simulink model "PV_WIND_BESS_SM_FIXED_R1"  (R2026a)
settings: Solver=ode14x  StopTime=3.2  FixedStep=25e-6  MaxStep=1e-5
InitFcn:
  | setup_v2_paths;init_grid_supported_integration;run(which('init_bess_vsm_r10.m'));
undefined symbols (not defined in the file): Base, Control, Converter, DiscIntNeverNeededParam, Drive, Filter, G, PMSG, V2, Wind
libraries: nesl_utility x50, ee_lib x43, fl_lib x25, simulink x5, sl_discontinuities x1
(part 1 of 4)
Description:
  | Three resources on 10 kV strong synchronous grid. Commissioning candidate only. BESS tie blocked. Wind interface delay 100 us; continuous wind dynamics retained.
settings Model: Creator=fakebob2004  LastModifiedBy=fakebob2004
settings SimscapeCC: SimscapeLogType=none

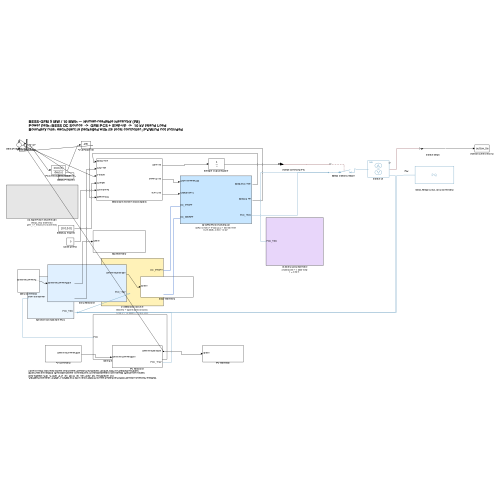
[thumbnail: Simulink's stored preview of the top-level diagram]
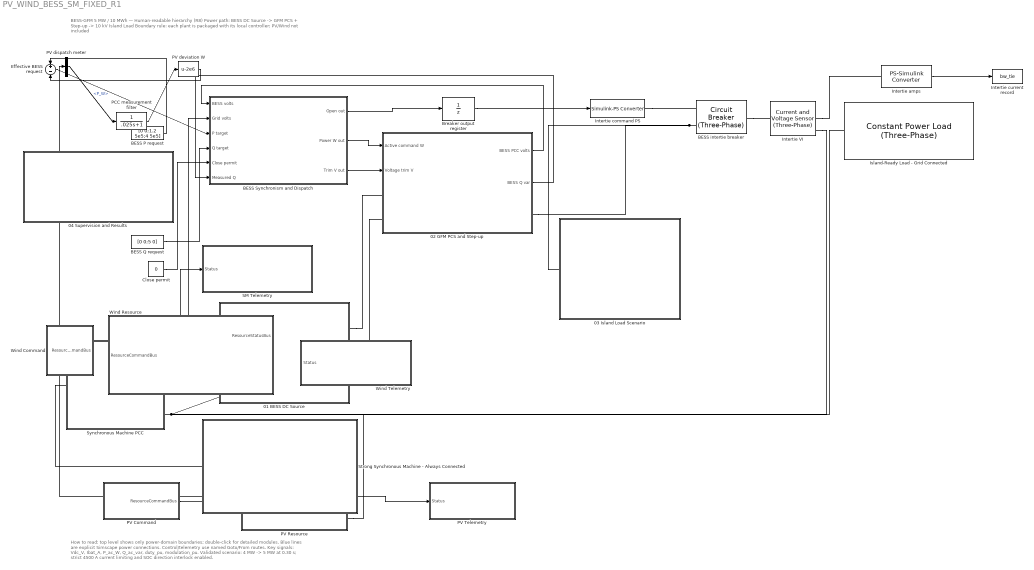
== system PV_WIND_BESS_SM_FIXED_R1 ==
  note: BESS-GFM 5 MW / 10 MWh — Human-readable hierarchy (R8)
      | Power path: BESS DC Source  ->  GFM PCS + Step-up  ->  10 kV Island Load
      | Boundary rule: each plant is packaged with its local controller; PV/Wind not included
  note: How to read: top level shows only power-domain boundaries; double-click for detailed modules.
      | Blue lines are explicit Simscape power connections. Control/telemetry use named Goto/From routes.
      | Key signals: Vdc_V, Ibat_A, P_ac_W, Q_ac_var, duty_pu, modulation_pu.
      | Validated scenario: 4 MW -> 5 MW at 0.30 s; strict 4500 A current limiting and SOC direction interlock enabled.
  01 BESS DC Source : Subsystem
      settings: AttributesFormatString=Battery + bidirectional DC/DC\n1200 V / 10 MWh -> 1500 Vdc
  02 GFM PCS and Step-up : Subsystem
      settings: AttributesFormatString=GFM control + PCS/LCL + transformer\n6.25 MVA, 0.69 / 10 kV
  03 Island Load Scenario : Subsystem
      settings: AttributesFormatString=4 MW base + 1 MW step\nt = 0.30 s
  04 Supervision and Results : Subsystem
      settings: AttributesFormatString=Read-only telemetry\ngfm_r7_result (15 channels)
  BESS P request : FromWorkspace  VariableName=[0 0;1.2 5e5;4 5e5]  Interpolate=off  OutputAfterFinalValue=Holding final value
  BESS Q request : FromWorkspace  VariableName=[0 0;5 0]  Interpolate=off  OutputAfterFinalValue=Holding final value
  BESS Synchronism and Dispatch : Subsystem
  BESS intertie breaker : ee_lib/Switches & Breakers/Circuit Breaker (Three-Phase)  port_option=ee.enum.threePhasePort.composite  control_port_option=ee.enum.controlport.ps  R_closed=0.001 Ohm  G_open=1e-6 1/Ohm  threshold=0.5 V  breaker_behavior=ee.enum.switches.breakerBehavior.zeroCrossingDisable  i_th=1e-8 A
  Breaker output register : UnitDelay  InitialCondition=1  SampleTime=.001
  Close permit : Constant  Value=0
  Effective BESS request : Sum  Inputs=+-
  Intertie VI : ee_lib/Sensors & Transducers/Current and Voltage Sensor (Three-Phase)  port_option=ee.enum.threePhasePort.composite  vMeasurementType=ee.enum.vmeasurement.ll  outputUnit=ee.enum.unit.si  SRated=100e6 A*V  VRated=24e3 V  I_specify=off  I_priority=None  I=[0, 0, 0] A  I_nominal_specify=off  I_nominal_value=1  I_nominal_unit=A  V_specify=off  V_priority=None  V=[0, 0, 0] V  V_nominal_specify=off  V_nominal_value=1  V_nominal_unit=V
  Intertie amps : nesl_utility/PS-Simulink Converter  PhysicalDomain=network_engine_domain  SubClassName=ps_output  LeftPortType=input  RightPortType=output  PseudoPeriodic=off  Frequencies=[]  VectorFormat=inherit  Unit=A  AffineConversion=off
  Intertie command PS : nesl_utility/Simulink-PS Converter  PhysicalDomain=network_engine_domain  SubClassName=ps_input  LeftPortType=input  RightPortType=output  PseudoPeriodic=off  Frequencies=[]  NoiseDistribution=none  NoiseParameters=[]  Unit=V  AffineConversion=off  FilteringAndDerivatives=zero  SimscapeFilterOrder=1  InputFilterTimeConstant=0.001  UdotUserProvided=0
  Intertie current record : ToWorkspace  VariableName=bw_tie  SaveFormat=Timeseries  SampleTime=-1
  Island-Ready Load - Grid Connected : ee_lib/Passive/Constant Power Load (Three-Phase)  port_option=ee.enum.threePhasePort.composite  FRated=50 Hz  active_power=5e6 W  reactive_power=1.5e6 V*A  Vline_rms_min=7000 V  tau=0.01 s  Vline_rms_ini=10000 V  Vang_ini=0 deg  gmin=1e-6 S
  PCC measurement filter : TransferFcn  Numerator=1  Denominator=[.025 1]
  PV Command : Subsystem
  PV Resource : Subsystem
  PV Telemetry : Subsystem
  PV deviation W : Bias  Bias=-2e6  SaturateOnIntegerOverflow=off
  PV dispatch meter : BusSelector  OutputSignals=P_W
  SM Telemetry : Subsystem
  Strong Synchronous Machine - Always Connected : Subsystem
  Synchronous Machine PCC : Subsystem
  Wind Command : Subsystem
  Wind Resource : Subsystem
  Wind Telemetry : Subsystem
  wires:
  02 GFM PCS and Step-up/1(BESS PCC volts) -> BESS Synchronism and Dispatch/1(BESS volts)
  02 GFM PCS and Step-up/2(BESS Q var) -> BESS Synchronism and Dispatch/6(Measured Q)
  BESS Synchronism and Dispatch/2(Power W out) -> 02 GFM PCS and Step-up/1(Active command W)
  Intertie amps/1 -> Intertie current record/1
  BESS Synchronism and Dispatch/1(Open out) -> Breaker output register/1
  Breaker output register/1 -> Intertie command PS/1
  Close permit/1 -> BESS Synchronism and Dispatch/5(Close permit)
  Synchronous Machine PCC/1(PCCMeasurementBus) -> SM Telemetry/1(Status)
  BESS Q request/1 -> BESS Synchronism and Dispatch/4(Q target)
  BESS Synchronism and Dispatch/3(Trim V out) -> 02 GFM PCS and Step-up/2(Voltage trim V)
  Synchronous Machine PCC/2(Phase volts) -> BESS Synchronism and Dispatch/2(Grid volts)
  PV Command/1(ResourceCommandBus) -> PV Resource/1(ResourceCommandBus)
  PV Resource/1(ResourceStatusBus) -> PV Telemetry/1(Status), PV dispatch meter/1
  PV dispatch meter/1 -> PCC measurement filter/1  "<P_W>"
  PCC measurement filter/1 -> PV deviation W/1
  PV deviation W/1 -> Effective BESS request/2
  BESS P request/1 -> Effective BESS request/1
  Effective BESS request/1 -> BESS Synchronism and Dispatch/3(P target)
  Wind Command/1(ResourceCommandBus) -> Wind Resource/1(ResourceCommandBus)
  Wind Resource/1(ResourceStatusBus) -> Wind Telemetry/1(Status)
  connections:
  Intertie VI/RConn2 -- Intertie amps/LConn1
  BESS intertie breaker/RConn1 -- Intertie VI/LConn1
  Intertie command PS/RConn1 -- BESS intertie breaker/LConn1
  01 BESS DC Source/RConn2 -- 02 GFM PCS and Step-up/LConn2
  Strong Synchronous Machine - Always Connected/LConn1 -- Synchronous Machine PCC/LConn1
  01 BESS DC Source/RConn1 -- 02 GFM PCS and Step-up/LConn1
  Intertie VI/RConn3 -- Island-Ready Load - Grid Connected/LConn1 -- PV Resource/RConn1 -- Synchronous Machine PCC/RConn1 -- Wind Resource/RConn1
  02 GFM PCS and Step-up/RConn1 -- 03 Island Load Scenario/LConn1 -- BESS intertie breaker/LConn2

== system PV_WIND_BESS_SM_FIXED_R1/01 BESS DC Source ==
  01 Battery and DC Link : Subsystem
      settings: AttributesFormatString=1200 V / 10 MWh\n1500 V DC link
  02 Bidirectional DC-DC Control : Subsystem
      settings: AttributesFormatString=Vdc PI: 10 Hz\nIbat PI: 300 Hz
  DC_Positive : PMIOPort  Side=Right  ConnectionType=Connection: foundation.electrical.electrical
  DC_Negative : PMIOPort  Port=2  Side=Right  ConnectionType=Connection: foundation.electrical.electrical
  connections:
  02 Bidirectional DC-DC Control/RConn1 -- 01 Battery and DC Link/LConn2
  01 Battery and DC Link/RConn2 -- DC_Negative/RConn1
  DC_Positive/RConn1 -- 01 Battery and DC Link/LConn1

== system PV_WIND_BESS_SM_FIXED_R1/02 GFM PCS and Step-up ==
  Active command W : Inport
  Voltage trim V : Inport  Port=2
  03 GFM Control and Limits : Subsystem
      settings: AttributesFormatString=P-f / Q-V / Virtual Z\nAC limit: 1.20 pu
  04 PCS Filter and Transformer : Subsystem
      settings: AttributesFormatString=6.25 MVA PCS + LCL\n0.69 / 10 kV transformer
  DC_Positive : PMIOPort  Side=Left  ConnectionType=Connection: foundation.electrical.electrical
  DC_Negative : PMIOPort  Port=2  Side=Left  ConnectionType=Connection: foundation.electrical.electrical
  PCC_10kV : PMIOPort  Port=3  Side=Right  ConnectionType=Connection: foundation.electrical.three_phase
  BESS PCC volts : Outport
  BESS Q var : Outport  Port=2
  wires:
  03 GFM Control and Limits/1(GFM modulation reference) -> 04 PCS Filter and Transformer/1(GFM modulation reference)
  04 PCS Filter and Transformer/1(PreSync PCC volts) -> BESS PCC volts/1
  04 PCS Filter and Transformer/2(Measured Q var) -> BESS Q var/1
  Active command W/1 -> 03 GFM Control and Limits/1(Active command W)
  Voltage trim V/1 -> 03 GFM Control and Limits/2(Voltage trim V)
  connections:
  04 PCS Filter and Transformer/RConn3 -- DC_Negative/RConn1
  04 PCS Filter and Transformer/RConn2 -- PCC_10kV/RConn1
  04 PCS Filter and Transformer/RConn1 -- DC_Positive/RConn1
  ?

== system PV_WIND_BESS_SM_FIXED_R1/03 Island Load Scenario ==
  Adjusted_Island_Load : ee_lib/Passive/Constant Power Load (Three-Phase)  port_option=ee.enum.threePhasePort.composite  FRated=G.f0_Hz Hz  active_power=1e4 W  reactive_power=0 V*A  Vline_rms_min=0.70*G.ac.Vll_high_V V  tau=0.01 s  Vline_rms_ini=1e-3 V  Vang_ini=0 deg  gmin=1e-6 S
  Damping neutral : ee_lib/Connectors & References/Grounded Neutral (Three-Phase)  port_option=ee.enum.threePhasePort.composite
  Feeder open request : MinMax  Function=max  Inputs=2
  Load_Step_Command : Step  Time=G.load.step_time_s  InitialValue=1  SampleTime=0
  Load_Step_to_PS : nesl_utility/Simulink-PS Converter  PhysicalDomain=network_engine_domain  SubClassName=ps_input  LeftPortType=input  RightPortType=output  PseudoPeriodic=off  Frequencies=[]  NoiseDistribution=none  NoiseParameters=[]  Unit=V  AffineConversion=off  FilteringAndDerivatives=zero  SimscapeFilterOrder=1  InputFilterTimeConstant=0.001  UdotUserProvided=0
  One_MW_Step_Load : ee_lib/Passive/Constant Power Load (Three-Phase)  port_option=ee.enum.threePhasePort.composite  FRated=G.f0_Hz Hz  active_power=G.load.step_P_W W  reactive_power=G.load.step_Q_var V*A  Vline_rms_min=0.70*G.ac.Vll_high_V V  tau=0.01 s  Vline_rms_ini=1e-3 V  Vang_ini=0 deg  gmin=1e-6 S
  PCC damping RC : ee_lib/Passive/RLC Assemblies/RLC (Three-Phase)  port_option=ee.enum.threePhasePort.composite  component_structure=ee.enum.rlc.structure.SeriesRC  R=10 Ohm  L=1e-3 H  C=1e-6 F  R_parasitic=0 Ohm  G_parasitic=0 1/Ohm  IL_specify=off  IL_priority=High  IL=[0, 0, 0] A  IL_nominal_specify=off  IL_nominal_value=1  IL_nominal_unit=A  VC_specify=off  VC_priority=High  VC=[0, 0, 0] V  VC_nominal_specify=off  VC_nominal_value=1  VC_nominal_unit=V
  Startup feeder hold : Step  Time=.12  InitialValue=1  FinalValue=0  SampleTime=0
  Step_Load_Breaker : ee_lib/Switches & Breakers/Circuit Breaker (Three-Phase)  port_option=ee.enum.threePhasePort.composite  control_port_option=ee.enum.controlport.ps  R_closed=0.001 Ohm  G_open=1e-6 1/Ohm  threshold=0.5 V  breaker_behavior=ee.enum.switches.breakerBehavior.zeroCrossingEnable  i_th=1e-8 A
  PCC_10kV : PMIOPort  Side=Left  ConnectionType=Connection: foundation.electrical.three_phase
  tag scope: R8_05_Island_Load_Scenario_p1_signal=global
  wires:
  Load_Step_Command/1 -> [R8_05_Island_Load_Scenario_p1_signal], Feeder open request/1  "step_breaker_cmd"
  Startup feeder hold/1 -> Feeder open request/2
  Feeder open request/1 -> Load_Step_to_PS/1
  connections:
  Step_Load_Breaker/RConn1 -- One_MW_Step_Load/LConn1
  PCC_10kV/RConn1 -- PCC damping RC/LConn1 -- Adjusted_Island_Load/LConn1 -- Step_Load_Breaker/LConn2
  Load_Step_to_PS/RConn1 -- Step_Load_Breaker/LConn1
  PCC damping RC/RConn1 -- Damping neutral/LConn1

== system PV_WIND_BESS_SM_FIXED_R1/04 Supervision and Results ==
  R7_Result_Mux : Mux  Inputs=15
  R7_Results : ToWorkspace  VariableName=gfm_r7_result  SampleTime=-1
  Time : Clock
  wires:
  [R8_05_Island_Load_Scenario_p1_signal] -> R7_Result_Mux/15
  [R8_03_GFM_Control_and_Limits_p7_signal] -> R7_Result_Mux/14
  R7_Result_Mux/1 -> R7_Results/1
  [R8_03_GFM_Control_and_Limits_p6_signal] -> R7_Result_Mux/13
  [R8_02_Bidirectional_DC_DC_Control_p3_signal] -> R7_Result_Mux/12
  [R8_02_Bidirectional_DC_DC_Control_p2_signal] -> R7_Result_Mux/11
  [R8_01_Battery_and_DC_Link_p3_signal] -> R7_Result_Mux/10
  [R8_03_GFM_Control_and_Limits_p3_signal] -> R7_Result_Mux/9
  [R8_01_Battery_and_DC_Link_p2_signal] -> R7_Result_Mux/8
  [R8_01_Battery_and_DC_Link_p1_signal] -> R7_Result_Mux/7
  [R8_01_Battery_and_DC_Link_p4_signal] -> R7_Result_Mux/6
  [R8_03_GFM_Control_and_Limits_p2_signal] -> R7_Result_Mux/5
  Time/1 -> R7_Result_Mux/1  "time_s"
  [R8_03_GFM_Control_and_Limits_p5_signal] -> R7_Result_Mux/4
  [R8_03_GFM_Control_and_Limits_p1_signal] -> R7_Result_Mux/3
  [R8_03_GFM_Control_and_Limits_p4_signal] -> R7_Result_Mux/2

== system PV_WIND_BESS_SM_FIXED_R1/BESS Synchronism and Dispatch ==
  BESS volts : Inport
  Grid volts : Inport  Port=2
  P target : Inport  Port=3
  Q target : Inport  Port=4
  Close permit : Inport  Port=5
  Measured Q : Inport  Port=6
  Inputs : Mux  Inputs=7
  Open : Fcn  Expr=u(1)
  Power W : Fcn  Expr=u(2)
  Record : ToWorkspace  VariableName=bw_sync  SaveFormat=Timeseries  SampleTime=-1
  Sample : ZeroOrderHold  SampleTime=.001
  State : UnitDelay  InitialCondition=zeros(9,1)  SampleTime=.001
  Synchrocheck and latch : MATLAB Function  TreatAsAtomicUnit=on
  Time : Clock
  Trim V : Fcn  Expr=u(3)
  Open out : Outport
  Power W out : Outport  Port=2
  Trim V out : Outport  Port=3
  wires:
  BESS volts/1 -> Inputs/1
  Grid volts/1 -> Inputs/2
  P target/1 -> Inputs/3
  Q target/1 -> Inputs/4
  Time/1 -> Inputs/5
  Close permit/1 -> Inputs/6
  Measured Q/1 -> Inputs/7
  Inputs/1 -> Sample/1
  Sample/1 -> Synchrocheck and latch/1(u)
  State/1 -> Synchrocheck and latch/2(z)
  Synchrocheck and latch/2(z1) -> State/1
  Synchrocheck and latch/1(y) -> Record/1, Open/1, Power W/1, Trim V/1
  Open/1 -> Open out/1
  Power W/1 -> Power W out/1
  Trim V/1 -> Trim V out/1

== system PV_WIND_BESS_SM_FIXED_R1/PV Command ==
  Command : BusCreator  Inputs=6  OutDataTypeStr=Bus: ResourceCommandBus
  Enable : Constant
  Mode : Constant  Value=0
  P Base : Constant  Value=2000000
  P Increment : Step  Time=2.1  FinalValue=1e6  SampleTime=0
  P Reference : Sum
  Q Reference : Step  Time=10  FinalValue=0  SampleTime=0
  V Reference : Constant  Value=690
  f Reference : Constant  Value=50
  ResourceCommandBus : Outport  OutDataTypeStr=Bus: ResourceCommandBus
  wires:
  Command/1 -> ResourceCommandBus/1
  Mode/1 -> Command/6  "mode"
  Enable/1 -> Command/5  "enable"
  f Reference/1 -> Command/4  "f_ref_Hz"
  V Reference/1 -> Command/3  "V_ref_V"
  Q Reference/1 -> Command/2  "Q_ref_var"
  P Reference/1 -> Command/1  "P_ref_W"
  P Increment/1 -> P Reference/2
  P Base/1 -> P Reference/1

== system PV_WIND_BESS_SM_FIXED_R1/PV Resource ==
  ResourceCommandBus : Inport  OutDataTypeStr=Bus: ResourceCommandBus
  01 PV Array : Subsystem
  02 MPPT Boost and DC Link : Subsystem
  03 Average Grid Converter : Subsystem
  04 Local GFL Control : Subsystem
  05 Filter Transformer and PCC : Subsystem
      settings: AttributesFormatString=independent filter + 0.69/10 kV transformer + PCC sensing
  Command Interface : Subsystem
  Resource Status : Subsystem
  PCC_10kV : PMIOPort  Side=Right  ConnectionType=Connection: foundation.electrical.three_phase
  ResourceStatusBus : Outport  OutDataTypeStr=Bus: ResourceStatusBus
  wires:
  Resource Status/1(Status) -> ResourceStatusBus/1
  Command Interface/3(mode) -> Resource Status/4(mode)
  04 Local GFL Control/2(controlData) -> Resource Status/3(controlData)
  04 Local GFL Control/1(modulationABC) -> 03 Average Grid Converter/1(modulationABC)
  02 MPPT Boost and DC Link/1(sourceData) -> Resource Status/2(sourceData), 04 Local GFL Control/3(sourceData)
  03 Average Grid Converter/1(converterCurrentABC) -> 04 Local GFL Control/2(converterCurrentABC)
  05 Filter Transformer and PCC/1(PCCMeasurementBus) -> Resource Status/1(PCC), 04 Local GFL Control/1(PCCMeasurementBus)
  01 PV Array/1(arrayVI) -> 02 MPPT Boost and DC Link/2(arrayVI)
  Command Interface/2(gridDispatch) -> 04 Local GFL Control/4(dispatch)
  Command Interface/1(sourceDispatch) -> 02 MPPT Boost and DC Link/1(dispatch)
  ResourceCommandBus/1 -> Command Interface/1(Command)
  connections:
  05 Filter Transformer and PCC/RConn1 -- PCC_10kV/RConn1
  03 Average Grid Converter/RConn1 -- 05 Filter Transformer and PCC/LConn1
  02 MPPT Boost and DC Link/RConn2 -- 03 Average Grid Converter/LConn2
  01 PV Array/RConn2 -- 02 MPPT Boost and DC Link/LConn2
  02 MPPT Boost and DC Link/RConn1 -- 03 Average Grid Converter/LConn1
  01 PV Array/RConn1 -- 02 MPPT Boost and DC Link/LConn1

== system PV_WIND_BESS_SM_FIXED_R1/PV Telemetry ==
  Status : Inport
  Fields : BusSelector  OutputSignals=P_W,Q_var,Vpcc_V,frequency_Hz,available_power_W,power_headroom_W,current_limit_factor,energy_state_pu,Vdc_V,control_mode,healthy
  Record : ToWorkspace  VariableName=integration_pv  SaveFormat=Timeseries  SampleTime=-1
  Vector : Mux  Inputs=11
  wires:
  Vector/1 -> Record/1
  Fields/11 -> Vector/11  "<healthy>"
  Fields/10 -> Vector/10  "<control_mode>"
  Fields/9 -> Vector/9  "<Vdc_V>"
  Fields/8 -> Vector/8  "<energy_state_pu>"
  Fields/7 -> Vector/7  "<current_limit_factor>"
  Fields/6 -> Vector/6  "<power_headroom_W>"
  Fields/5 -> Vector/5  "<available_power_W>"
  Fields/4 -> Vector/4  "<frequency_Hz>"
  Fields/3 -> Vector/3  "<Vpcc_V>"
  Fields/2 -> Vector/2  "<Q_var>"
  Fields/1 -> Vector/1  "<P_W>"
  Status/1 -> Fields/1

== system PV_WIND_BESS_SM_FIXED_R1/SM Telemetry ==
  Status : Inport
  Fields : BusSelector  OutputSignals=P_W,Q_var,Vll_rms_V
  Record : ToWorkspace  VariableName=integration_sm  SaveFormat=Timeseries  SampleTime=-1
  Vector : Mux  Inputs=3
  wires:
  Vector/1 -> Record/1
  Fields/3 -> Vector/3  "<Vll_rms_V>"
  Fields/2 -> Vector/2  "<Q_var>"
  Fields/1 -> Vector/1  "<P_W>"
  Status/1 -> Fields/1

== system PV_WIND_BESS_SM_FIXED_R1/Strong Synchronous Machine - Always Connected ==
  Excitation : Constant  Value=1e4*sqrt(2/3)
  Excitation PS : nesl_utility/Simulink-PS Converter  PhysicalDomain=network_engine_domain  SubClassName=ps_input  LeftPortType=input  RightPortType=output  PseudoPeriodic=off  Frequencies=[]  NoiseDistribution=none  NoiseParameters=[]  Unit=V  AffineConversion=off  FilteringAndDerivatives=zero  SimscapeFilterOrder=1  InputFilterTimeConstant=0.001  UdotUserProvided=0
  Governor Speed : Step  Time=10  InitialValue=2*pi*50  FinalValue=2*pi*50  SampleTime=0
  Ideal Governor : fl_lib/Mechanical/Mechanical Sources/Ideal Angular Velocity Source
  Machine Measurements : nesl_utility/PS-Simulink Converter  PhysicalDomain=network_engine_domain  SubClassName=ps_output  LeftPortType=input  RightPortType=output  PseudoPeriodic=off  Frequencies=[]  VectorFormat=inherit  Unit=1  AffineConversion=off
  Machine Record : ToWorkspace  VariableName=integration_machine  SaveFormat=Timeseries  SampleTime=-1
  Mechanical Reference : fl_lib/Mechanical/Rotational Elements/Mechanical Rotational Reference
  Neutral : fl_lib/Electrical/Electrical Elements/Electrical Reference
  Speed PS : nesl_utility/Simulink-PS Converter  PhysicalDomain=network_engine_domain  SubClassName=ps_input  LeftPortType=input  RightPortType=output  PseudoPeriodic=off  Frequencies=[]  NoiseDistribution=none  NoiseParameters=[]  Unit=rad/s  AffineConversion=off  FilteringAndDerivatives=zero  SimscapeFilterOrder=1  InputFilterTimeConstant=0.001  UdotUserProvided=0
  Synchronous Machine : ee_lib/Electromechanical/Synchronous/Simplified Synchronous Machine  port_option=ee.enum.threePhasePort.composite  SRated=100e6 A*V  VRated=10e3 V  FRated=50 Hz  nPolePairs=1  param_unit=ee.enum.unit.si  R_si=0.01 Ohm  L_si=0.001 H  R_pu=0.05  L_pu=0.3  initialization_option=ee.enum.sm.initialization.electrical  source_type=ee.enum.sm.load_flow_source_type.Swing  Vmag0=10e3 V  Vang0=0 deg  Pt0=5e6 A*V  Qt0=1.5e6 A*V  minimum_pu=0.95  phase_search_range=[-inf, inf] deg  gmin=1e-6 S  connection_option=ee.enum.Connection.wye  angular_position_diff_specify=off  angular_position_diff_priority=None  angular_position_diff=0 rad  angular_position_diff_nominal_specify=off  angular_position_diff_nominal_value=1  angular_position_diff_nominal_unit=rad  pu_psid_specify=off  pu_psid_priority=None  pu_psid=0  pu_psid_nominal_specify=off  pu_psid_nominal_value=1  pu_psid_nominal_unit=1  pu_psiq_specify=off  pu_psiq_priority=None  pu_psiq=0  pu_psiq_nominal_specify=off  pu_psiq_nominal_value=1  pu_psiq_nominal_unit=1  pu_psi0_specify=off  pu_psi0_priority=None  pu_psi0=0  pu_psi0_nominal_specify=off  pu_psi0_nominal_value=1  pu_psi0_nominal_unit=1  angular_torque_specify=off  angular_torque_priority=None  angular_torque=0 N*m  angular_torque_nominal_specify=off  angular_torque_nominal_value=1  angular_torque_nominal_unit=N*m  Tmeas=298.15 K  alpha=3.93e-3 1/K  stator_thermal_mass=100 J/K  rotor_thermal_mass=200 J/K  temperatureA_specify=off  temperatureA_priority=High  temperatureA=25 degC  temperatureA_nominal_specify=off  temperatureA_nominal_value=1  temperatureA_nominal_unit=degC  temperatureB_specify=off  temperatureB_priority=High  temperatureB=25 degC  temperatureB_nominal_specify=off  temperatureB_nominal_value=1  temperatureB_nominal_unit=degC  temperatureC_specify=off  temperatureC_priority=High  temperatureC=25 degC  temperatureC_nominal_specify=off  temperatureC_nominal_value=1  temperatureC_nominal_unit=degC  temperatureR_specify=off  temperatureR_priority=High  temperatureR=25 degC  temperatureR_nominal_specify=off  temperatureR_nominal_value=1  temperatureR_nominal_unit=degC
  PCC : PMIOPort  Side=Left  ConnectionType=Connection: foundation.electrical.three_phase
  wires:
  Governor Speed/1 -> Speed PS/1
  Excitation/1 -> Excitation PS/1
  Machine Measurements/1 -> Machine Record/1
  connections:
  PCC/RConn1 -- Synchronous Machine/RConn2
  Synchronous Machine/RConn3 -- Neutral/LConn1
  Excitation PS/RConn1 -- Synchronous Machine/LConn1
  Speed PS/RConn1 -- Ideal Governor/RConn1
  Ideal Governor/LConn1 -- Synchronous Machine/LConn2
  Mechanical Reference/LConn1 -- Ideal Governor/RConn2 -- Synchronous Machine/LConn3
  Synchronous Machine/RConn1 -- Machine Measurements/LConn1

== system PV_WIND_BESS_SM_FIXED_R1/Synchronous Machine PCC ==
  Local PCC Voltage Record : ToWorkspace  VariableName=integration_bus_vabc  SaveFormat=Timeseries  SampleTime=-1
  Nominal Frequency : Constant  Value=V2.PV.rating.f_Hz
  P to Simulink : nesl_utility/PS-Simulink Converter  PhysicalDomain=network_engine_domain  SubClassName=ps_output  LeftPortType=input  RightPortType=output  PseudoPeriodic=off  Frequencies=[]  VectorFormat=inherit  Unit=W  AffineConversion=off
  PCC Measurement : BusCreator  Inputs=6  OutDataTypeStr=Bus: PCCMeasurementBus
  PCC Power Sensor : ee_lib/Sensors & Transducers/Power Sensor (Three-Phase)  port_option=ee.enum.threePhasePort.composite  load_type=ee.enum.passive.type_balanced.balanced  f0=60 Hz
  PCC VI Sensor : ee_lib/Sensors & Transducers/Current and Voltage Sensor (Three-Phase)  port_option=ee.enum.threePhasePort.composite  vMeasurementType=ee.enum.vmeasurement.lg  outputUnit=ee.enum.unit.si  SRated=100e6 A*V  VRated=24e3 V  I_specify=off  I_priority=None  I=[0, 0, 0] A  I_nominal_specify=off  I_nominal_value=1  I_nominal_unit=A  V_specify=off  V_priority=None  V=[0, 0, 0] V  V_nominal_specify=off  V_nominal_value=1  V_nominal_unit=V
  Q to Simulink : nesl_utility/PS-Simulink Converter  PhysicalDomain=network_engine_domain  SubClassName=ps_output  LeftPortType=input  RightPortType=output  PseudoPeriodic=off  Frequencies=[]  VectorFormat=inherit  Unit=W  AffineConversion=off
  Vll RMS : Fcn  Expr=sqrt(u(1)^2+u(2)^2+u(3)^2)
  iabc to Simulink : nesl_utility/PS-Simulink Converter  PhysicalDomain=network_engine_domain  SubClassName=ps_output  LeftPortType=input  RightPortType=output  PseudoPeriodic=off  Frequencies=[]  VectorFormat=inherit  Unit=A  AffineConversion=off
  vabc to Simulink : nesl_utility/PS-Simulink Converter  PhysicalDomain=network_engine_domain  SubClassName=ps_output  LeftPortType=input  RightPortType=output  PseudoPeriodic=off  Frequencies=[]  VectorFormat=inherit  Unit=V  AffineConversion=off
  From Transformer : PMIOPort  Side=Left  ConnectionType=Connection: foundation.electrical.three_phase
  PCC_10kV : PMIOPort  Port=2  Side=Right  ConnectionType=Connection: foundation.electrical.three_phase
  PCCMeasurementBus : Outport  OutDataTypeStr=Bus: PCCMeasurementBus
  Phase volts : Outport  Port=2
  wires:
  PCC Measurement/1 -> PCCMeasurementBus/1
  Nominal Frequency/1 -> PCC Measurement/6  "frequency_Hz"
  Vll RMS/1 -> PCC Measurement/5  "Vll_rms_V"
  Q to Simulink/1 -> PCC Measurement/4  "Q_var"
  P to Simulink/1 -> PCC Measurement/3  "P_W"
  iabc to Simulink/1 -> PCC Measurement/2  "iabc_A"
  vabc to Simulink/1 -> PCC Measurement/1, Local PCC Voltage Record/1, Vll RMS/1, Phase volts/1  "vabc_V"
  connections:
  PCC Power Sensor/LConn3 -- Q to Simulink/LConn1
  PCC Power Sensor/LConn2 -- P to Simulink/LConn1
  PCC VI Sensor/RConn2 -- iabc to Simulink/LConn1
  PCC VI Sensor/RConn1 -- vabc to Simulink/LConn1
  PCC Power Sensor/RConn1 -- PCC_10kV/RConn1
  PCC VI Sensor/RConn3 -- PCC Power Sensor/LConn1
  From Transformer/RConn1 -- PCC VI Sensor/LConn1

== system PV_WIND_BESS_SM_FIXED_R1/Wind Command ==
  Command : BusCreator  Inputs=6  OutDataTypeStr=Bus: ResourceCommandBus
  Enable : Constant
  Mode : Constant  Value=0
  P Base : Constant  Value=2e6
  P Increment : Step  Time=10  FinalValue=0  SampleTime=0
  P Reference : Sum
  Q Reference : Step  Time=10  FinalValue=0  SampleTime=0
  V Reference : Constant  Value=690
  f Reference : Constant  Value=50
  ResourceCommandBus : Outport  OutDataTypeStr=Bus: ResourceCommandBus
  wires:
  Command/1 -> ResourceCommandBus/1
  Mode/1 -> Command/6  "mode"
  Enable/1 -> Command/5  "enable"
  f Reference/1 -> Command/4  "f_ref_Hz"
  V Reference/1 -> Command/3  "V_ref_V"
  Q Reference/1 -> Command/2  "Q_ref_var"
  P Reference/1 -> Command/1  "P_ref_W"
  P Increment/1 -> P Reference/2
  P Base/1 -> P Reference/1

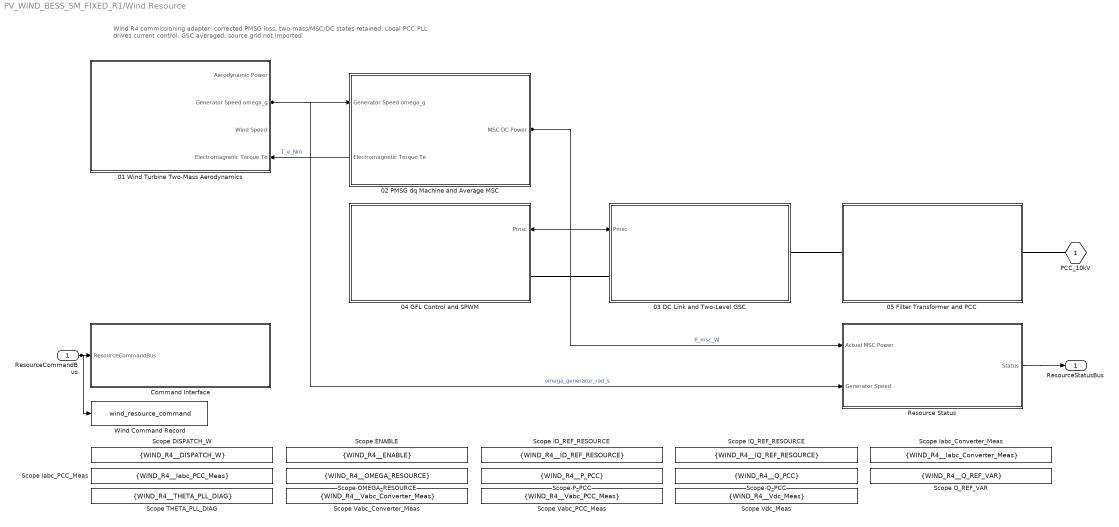
== system PV_WIND_BESS_SM_FIXED_R1/Wind Resource ==
  note: Wind R4 commissioning adapter: corrected PMSG loss, two-mass/MSC/DC states retained. Local PCC PLL drives current control. GSC averaged; source grid not imported.
  ResourceCommandBus : Inport  OutDataTypeStr=Bus: ResourceCommandBus
  01 Wind Turbine Two-Mass Aerodynamics : Subsystem
      settings: PortSchema="{\"entries\":[{\"content\":{\"sides\":[{\"content\":{},\"type\":\"ConnectorPlacement.EquallySpacedRectSide\",\"uuid\":\"d2e99250-fb32-457d-ac2c-6cda9d3cb83e\"},{\"content\":{\"connectorIds\":[\"Out1\",\"Out2\",\"Out3\",\"In1\"],\"side\":\"RIGHT\"},\"type\":\"ConnectorPlacement.EquallySpacedRectSide\",\"uuid\":\"4ed32267-e8b5-4207-a2ca-ef88d31c29b8\"},{\"content\":{\"side\":\"TOP\"},\"type\":\"ConnectorPlacement.EquallySpacedRectSide\",\"uuid\":\"49cb7178-688c-4425-86b9-2e86b87a92d2\"},{\"content\":{\"side\":\"BOTTOM\"},\"type\":\"ConnectorPlacement.EquallySpacedRectSide\",\"uuid\":\"608adf3d-9984-4c8c-8c51-00622b75c623\"}]},\"type\":\"ConnectorPlacement.EquallySpacedConnector\",\"uuid\":\"34aeb2da-84b2-49da-b11b-ab9d51671e98\"}],\"packageUris\":[\"http://schema.mathworks.com/mf0/Connector/R2020b\"],\"version\":\"1.0\"}"
  02 PMSG dq Machine and Average MSC : Subsystem
      settings: PortSchema="{\"entries\":[{\"content\":{\"sides\":[{\"content\":{\"connectorIds\":[\"In1\",\"Out1\"]},\"type\":\"ConnectorPlacement.EquallySpacedRectSide\",\"uuid\":\"48609cb7-5ec2-40c8-9ad6-e417a7f110fc\"},{\"content\":{\"connectorIds\":[\"Out2\"],\"side\":\"RIGHT\"},\"type\":\"ConnectorPlacement.EquallySpacedRectSide\",\"uuid\":\"fe5978ba-7578-46e7-b8bd-8d766a317898\"},{\"content\":{\"side\":\"TOP\"},\"type\":\"ConnectorPlacement.EquallySpacedRectSide\",\"uuid\":\"e50b8460-8f11-49ca-af82-a50e0a9897ac\"},{\"content\":{\"side\":\"BOTTOM\"},\"type\":\"ConnectorPlacement.EquallySpacedRectSide\",\"uuid\":\"e858deaf-0aa3-40bd-b11b-e0cbf70df614\"}]},\"type\":\"ConnectorPlacement.EquallySpacedConnector\",\"uuid\":\"52c7dc97-51f1-4b4e-ac97-f0f7de231d0c\"}],\"packageUris\":[\"http://schema.mathworks.com/mf0/Connector/R2020b\"],\"version\":\"1.0\"}"
  03 DC Link and Two-Level GSC : Subsystem
  04 GFL Control and SPWM : Subsystem
      settings: PortSchema="{\"entries\":[{\"content\":{\"sides\":[{\"content\":{},\"type\":\"ConnectorPlacement.EquallySpacedRectSide\",\"uuid\":\"789c4a44-46fc-465a-8542-50ccb2941023\"},{\"content\":{\"connectorIds\":[\"In1\",\"RConn1\"],\"side\":\"RIGHT\"},\"type\":\"ConnectorPlacement.EquallySpacedRectSide\",\"uuid\":\"a82b7ba7-9d1b-4671-ba15-c7f8930ba494\"},{\"content\":{\"side\":\"TOP\"},\"type\":\"ConnectorPlacement.EquallySpacedRectSide\",\"uuid\":\"e4af03d8-b6a4-4af9-a989-7508e05466ea\"},{\"content\":{\"side\":\"BOTTOM\"},\"type\":\"ConnectorPlacement.EquallySpacedRectSide\",\"uuid\":\"c53f6650-4639-4f00-bd86-9fb4ea7f36eb\"}]},\"type\":\"ConnectorPlacement.EquallySpacedConnector\",\"uuid\":\"b3a75c1a-8bf0-4d48-a914-c2377b7f5048\"}],\"packageUris\":[\"http://schema.mathworks.com/mf0/Connector/R2020b\"],\"version\":\"1.0\"}"
  05 Filter Transformer and PCC : Subsystem
  Command Interface : Subsystem
  Resource Status : Subsystem
  Scope DISPATCH_W : GotoTagVisibility  GotoTag=WIND_R4__DISPATCH_W
  Scope ENABLE : GotoTagVisibility  GotoTag=WIND_R4__ENABLE
  Scope ID_REF_RESOURCE : GotoTagVisibility  GotoTag=WIND_R4__ID_REF_RESOURCE
  Scope IQ_REF_RESOURCE : GotoTagVisibility  GotoTag=WIND_R4__IQ_REF_RESOURCE
  Scope Iabc_Converter_Meas : GotoTagVisibility  GotoTag=WIND_R4__Iabc_Converter_Meas
  Scope Iabc_PCC_Meas : GotoTagVisibility  GotoTag=WIND_R4__Iabc_PCC_Meas
  Scope OMEGA_RESOURCE : GotoTagVisibility  GotoTag=WIND_R4__OMEGA_RESOURCE
  Scope P_PCC : GotoTagVisibility  GotoTag=WIND_R4__P_PCC
  Scope Q_PCC : GotoTagVisibility  GotoTag=WIND_R4__Q_PCC
  Scope Q_REF_VAR : GotoTagVisibility  GotoTag=WIND_R4__Q_REF_VAR
  Scope THETA_PLL_DIAG : GotoTagVisibility  GotoTag=WIND_R4__THETA_PLL_DIAG
  Scope Vabc_Converter_Meas : GotoTagVisibility  GotoTag=WIND_R4__Vabc_Converter_Meas
  Scope Vabc_PCC_Meas : GotoTagVisibility  GotoTag=WIND_R4__Vabc_PCC_Meas
  Scope Vdc_Meas : GotoTagVisibility  GotoTag=WIND_R4__Vdc_Meas
  Wind Command Record : ToWorkspace  VariableName=wind_resource_command  SaveFormat=Timeseries  SampleTime=-1
  PCC_10kV : PMIOPort  Side=Right  ConnectionType=Connection: foundation.electrical.three_phase
  ResourceStatusBus : Outport  OutDataTypeStr=Bus: ResourceStatusBus
  wires:
  Resource Status/1(Status) -> ResourceStatusBus/1
  ResourceCommandBus/1 -> Wind Command Record/1, Command Interface/1(ResourceCommandBus)
  02 PMSG dq Machine and Average MSC/2(MSC DC Power) -> Resource Status/1(Actual MSC Power), 04 GFL Control and SPWM/1(Pmsc), 03 DC Link and Two-Level GSC/1(Pmsc)  "P_msc_W"
  02 PMSG dq Machine and Average MSC/1(Electromagnetic Torque Te) -> 01 Wind Turbine Two-Mass Aerodynamics/1(Electromagnetic Torque Te)  "T_e_Nm"
  01 Wind Turbine Two-Mass Aerodynamics/2(Generator Speed omega_g) -> Resource Status/2(Generator Speed), 02 PMSG dq Machine and Average MSC/1(Generator Speed omega_g)  "omega_generator_rad_s"
  connections:
  05 Filter Transformer and PCC/RConn1 -- PCC_10kV/RConn1
  03 DC Link and Two-Level GSC/RConn1 -- 05 Filter Transformer and PCC/LConn1
  04 GFL Control and SPWM/RConn1 -- 03 DC Link and Two-Level GSC/LConn1

== system PV_WIND_BESS_SM_FIXED_R1/Wind Telemetry ==
  Status : Inport
  Fields : BusSelector  OutputSignals=P_W,Q_var,Vpcc_V,frequency_Hz,available_power_W,power_headroom_W,current_limit_factor,energy_state_pu,Vdc_V,control_mode,healthy
  Record : ToWorkspace  VariableName=integration_wind  SaveFormat=Timeseries  SampleTime=-1
  Vector : Mux  Inputs=11
  wires:
  Vector/1 -> Record/1
  Fields/11 -> Vector/11  "<healthy>"
  Fields/10 -> Vector/10  "<control_mode>"
  Fields/9 -> Vector/9  "<Vdc_V>"
  Fields/8 -> Vector/8  "<energy_state_pu>"
  Fields/7 -> Vector/7  "<current_limit_factor>"
  Fields/6 -> Vector/6  "<power_headroom_W>"
  Fields/5 -> Vector/5  "<available_power_W>"
  Fields/4 -> Vector/4  "<frequency_Hz>"
  Fields/3 -> Vector/3  "<Vpcc_V>"
  Fields/2 -> Vector/2  "<Q_var>"
  Fields/1 -> Vector/1  "<P_W>"
  Status/1 -> Fields/1

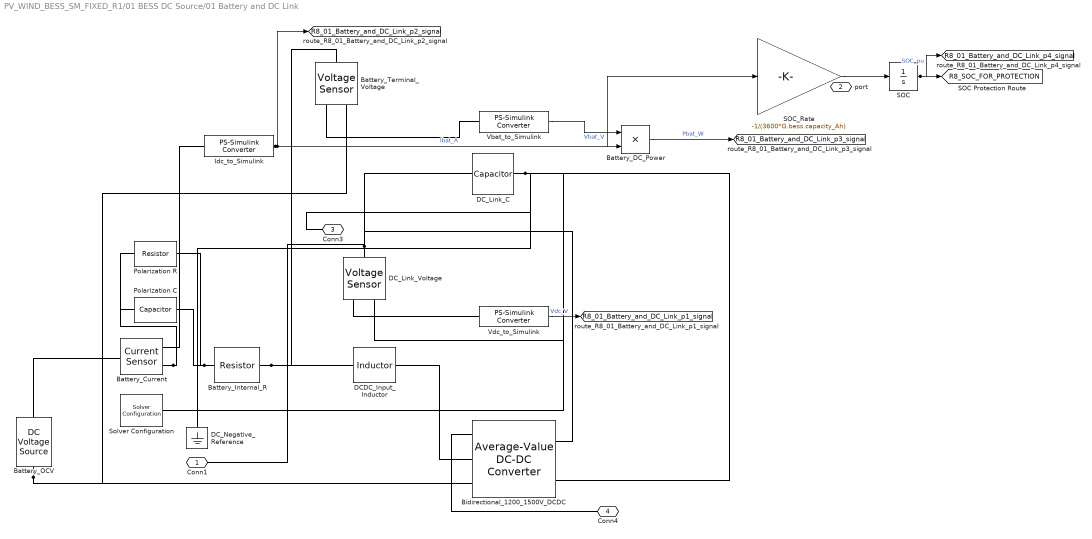
== system PV_WIND_BESS_SM_FIXED_R1/01 BESS DC Source/01 Battery and DC Link ==
  Battery_Current : fl_lib/Electrical/Electrical Sensors/Current Sensor
  Battery_DC_Power : Product
  Battery_Internal_R : fl_lib/Electrical/Electrical Elements/Resistor  R=G.r9.R0 Ohm  i_specify=off  i_priority=None  i=0 A  i_nominal_specify=off  i_nominal_value=1  i_nominal_unit=A  v_specify=off  v_priority=None  v=0 V  v_nominal_specify=off  v_nominal_value=1  v_nominal_unit=V
  Battery_OCV : fl_lib/Electrical/Electrical Sources/DC Voltage Source  v0=G.dc.Vbattery_V V
  Battery_Terminal_Voltage : fl_lib/Electrical/Electrical Sensors/Voltage Sensor
  Bidirectional_1200_1500V_DCDC : ee_lib/Semiconductors & Converters/Converters/Average-Value DC-DC Converter  implementation_option=ee.enum.converters.implementation.behavioral  converter_type=ee.enum.converters.dcdctype.buckboost  control_option=ee.enum.converters.controlinput.dutycycle  efficiency_option=ee.enum.converters.efficiency.constant  efficiency_fixed=G.dc.dcdc_efficiency_pct  i_vec=[0, 2, 5] A  efficiency_vec=[90, 95, 98]  Lf=1e-6 H  Rl=0 Ohm  Cf=1e-7 F  Rc=1e-6 Ohm  iL_specify=off  iL_priority=High  iL=0 A  iL_nominal_specify=off  iL_nominal_value=1  iL_nominal_unit=A  vc_specify=off  vc_priority=High  vc=0 V  vc_nominal_specify=off  vc_nominal_value=1  vc_nominal_unit=V
  DCDC_Input_Inductor : fl_lib/Electrical/Electrical Elements/Inductor  l=G.dcdc.L_H H  r=0 Ohm  g=1e-9 1/Ohm  i_specify=on  i_priority=None  i=G.dcdc.Iref_initial_A A  i_nominal_specify=off  i_nominal_value=1  i_nominal_unit=A  v_specify=off  v_priority=None  v=0 V  v_nominal_specify=off  v_nominal_value=1  v_nominal_unit=V  i_L_specify=off  i_L_priority=High  i_L=0 A  i_L_nominal_specify=off  i_L_nominal_value=1  i_L_nominal_unit=A
  DC_Link_C : fl_lib/Electrical/Electrical Elements/Capacitor  c=G.dc.Cdc_F F  r=1e-6 Ohm  g=0 1/Ohm  i_specify=off  i_priority=None  i=0 A  i_nominal_specify=off  i_nominal_value=1  i_nominal_unit=A  v_specify=off  v_priority=None  v=0 V  v_nominal_specify=off  v_nominal_value=1  v_nominal_unit=V  vc_specify=on  vc_priority=High  vc=G.dc.Vdc_ref_V V  vc_nominal_specify=off  vc_nominal_value=1  vc_nominal_unit=V
  DC_Link_Voltage : fl_lib/Electrical/Electrical Sensors/Voltage Sensor
  DC_Negative_Reference : fl_lib/Electrical/Electrical Elements/Electrical Reference
  Idc_to_Simulink : nesl_utility/PS-Simulink Converter  PhysicalDomain=network_engine_domain  SubClassName=ps_output  LeftPortType=input  RightPortType=output  PseudoPeriodic=off  Frequencies=[]  VectorFormat=inherit  Unit=A  AffineConversion=off
  Polarization C : fl_lib/Electrical/Electrical Elements/Capacitor  c=G.r9.tau/G.r9.Rp F  r=1e-6 Ohm  g=0 1/Ohm  i_specify=off  i_priority=None  i=0 A  i_nominal_specify=off  i_nominal_value=1  i_nominal_unit=A  v_specify=off  v_priority=None  v=0 V  v_nominal_specify=off  v_nominal_value=1  v_nominal_unit=V  vc_specify=on  vc_priority=High  vc=0 V  vc_nominal_specify=off  vc_nominal_value=1  vc_nominal_unit=V
  Polarization R : fl_lib/Electrical/Electrical Elements/Resistor  R=G.r9.Rp Ohm  i_specify=off  i_priority=None  i=0 A  i_nominal_specify=off  i_nominal_value=1  i_nominal_unit=A  v_specify=off  v_priority=None  v=0 V  v_nominal_specify=off  v_nominal_value=1  v_nominal_unit=V
  SOC : Integrator  InitialCondition=G.bess.SOC0  LimitOutput=on  UpperSaturationLimit=G.bess.SOC_max  LowerSaturationLimit=G.bess.SOC_min
  SOC_Rate : Gain  Gain=-1/(3600*G.bess.capacity_Ah)
  Solver Configuration : nesl_utility/Solver Configuration  PhysicalDomain=network_engine_domain  SubClassName=solver  LeftPortType=input  RightPortType=generic  Tones=[]  Harmonics=[]  SimulateNoise=off  Profile=off  UseLocalSampling=off  EnableSwitchedLinearOptims=on  FrequencyDomain=off  UseCCode=off  RelTol=0.001  AbsTol=0.001  MinStep=1e-09  ToWorkspace=off  RevertToSquareIcSolve=off  NumHomotopyIterations=100  PhasorMode=off  PhasorModeNumHarmonics=1  ConsistencySolver=NEWTON_XTOL_AFTER_FTOL  CanonicalOrdering=CANONICAL  OptimizeIntermediates=OPTIMIZED  IndexReductionMethod=DerivativeReplacement  DoDC=off  ResidualTolerance=1e-09  ConsistencyTolSource=GLOBAL  ConsistencyAbsTol=0.001  ConsistencyRelTol=0.001  ConsistencyTolFactor=0.001  UseLocalSolver=on  LocalSolverChoice=NE_BACKWARD_EULER_ADVANCER  ResolveIndetEquations=on  FunctionEvalNumThread=1  LocalSolverSampleTime=25e-6  DoFixedCost=off  MaxNonlinIter=3  MaxModeIter=2  ComputeImpulses=off  ImpulseIterations=2  LinearAlgebra=auto  LinearAlgebraNumThread=0  EquationFormulation=NE_TIME_EF  DelaysMemoryBudget=1024  AutomaticFiltering=on  FilteringTimeConstant=0.001  PartitionStorageMethod=AS_NEEDED  PartitionMemoryBudget=1024  PartitionMethod=ROBUST  MultibodyUseLocalSolver=off  MultibodyLocalSolverChoice=ODE1  MultibodyLocalSolverSampleTime=0.001
  Vbat_to_Simulink : nesl_utility/PS-Simulink Converter  PhysicalDomain=network_engine_domain  SubClassName=ps_output  LeftPortType=input  RightPortType=output  PseudoPeriodic=off  Frequencies=[]  VectorFormat=inherit  Unit=V  AffineConversion=off
  Vdc_to_Simulink : nesl_utility/PS-Simulink Converter  PhysicalDomain=network_engine_domain  SubClassName=ps_output  LeftPortType=input  RightPortType=output  PseudoPeriodic=off  Frequencies=[]  VectorFormat=inherit  Unit=V  AffineConversion=off
  Conn1 : PMIOPort  Side=Left
  port : PMIOPort  Port=2  Side=Right
  Conn3 : PMIOPort  Port=3  Side=Right
  Conn4 : PMIOPort  Port=4  Side=Left
  tag scope: R8_01_Battery_and_DC_Link_p1_signal=global, R8_01_Battery_and_DC_Link_p2_signal=global, R8_01_Battery_and_DC_Link_p3_signal=global, R8_01_Battery_and_DC_Link_p4_signal=global, R8_SOC_FOR_PROTECTION=global
  wires:
  SOC/1 -> [R8_01_Battery_and_DC_Link_p4_signal], [R8_SOC_FOR_PROTECTION]  "SOC_pu"
  Battery_DC_Power/1 -> [R8_01_Battery_and_DC_Link_p3_signal]  "Pbat_W"
  Vbat_to_Simulink/1 -> Battery_DC_Power/1  "Vbat_V"
  Vdc_to_Simulink/1 -> [R8_01_Battery_and_DC_Link_p1_signal]  "Vdc_V"
  SOC_Rate/1 -> SOC/1
  Idc_to_Simulink/1 -> [R8_01_Battery_and_DC_Link_p2_signal], Battery_DC_Power/2, SOC_Rate/1  "Ibat_A"
  connections:
  Conn4/RConn1 -- Bidirectional_1200_1500V_DCDC/LConn1
  DC_Link_Voltage/LConn1 -- Bidirectional_1200_1500V_DCDC/RConn1 -- DC_Link_C/LConn1 -- Conn1/RConn1
  Battery_Terminal_Voltage/RConn1 -- Vbat_to_Simulink/LConn1
  DC_Link_Voltage/RConn1 -- Vdc_to_Simulink/LConn1
  Battery_Internal_R/RConn1 -- DCDC_Input_Inductor/LConn1 -- Battery_Terminal_Voltage/LConn1
  DCDC_Input_Inductor/RConn1 -- Bidirectional_1200_1500V_DCDC/LConn2
  Battery_Current/RConn1 -- Idc_to_Simulink/LConn1
  Battery_OCV/LConn1 -- Battery_Current/LConn1
  DC_Negative_Reference/LConn1 -- DC_Link_C/RConn1 -- Bidirectional_1200_1500V_DCDC/RConn2 -- DC_Link_Voltage/RConn2 -- Conn3/RConn1 -- Solver Configuration/RConn1
  Battery_OCV/RConn1 -- Battery_Terminal_Voltage/RConn2 -- Bidirectional_1200_1500V_DCDC/LConn3
  Polarization R/LConn1 -- Battery_Current/RConn2 -- Polarization C/LConn1
  Battery_Internal_R/LConn1 -- Polarization R/RConn1 -- Polarization C/RConn1

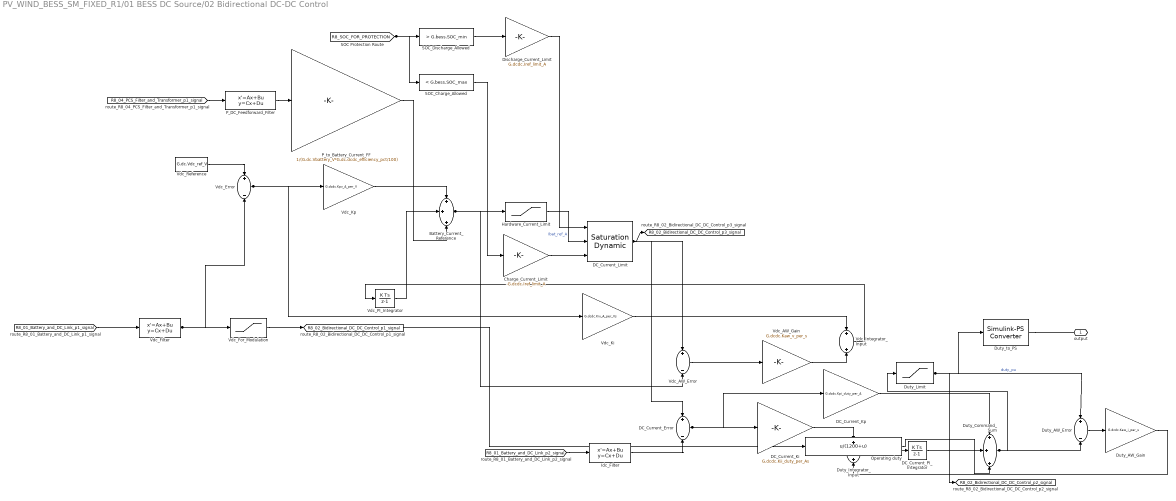
== system PV_WIND_BESS_SM_FIXED_R1/01 BESS DC Source/02 Bidirectional DC-DC Control ==
  Battery_Current_Reference : Sum  Inputs=+++
  Charge_Current_Limit : Gain  Gain=-G.dcdc.Iref_limit_A
  DC_Current_Error : Sum  Inputs=+-
  DC_Current_Ki : Gain  Gain=G.dcdc.Kii_duty_per_As
  DC_Current_Kp : Gain  Gain=G.dcdc.Kpi_duty_per_A
  DC_Current_Limit : sl_discontinuities/Saturation Dynamic  OutMin=[]  OutMax=[]  OutDataTypeStr=Inherit: Same as second input  OutDataType=fixdt(1, 16)  OutScaling=2^-10  DoSatur=off
      settings: LibrarySourceBlock=|
      | simulink/Discontinuities/Saturation
      | Dynamic
  DC_Current_PI_Integrator : DiscreteIntegrator  SampleTime=100e-6  ICPrevOutput=DiscIntNeverNeededParam  ICPrevScaledInput=DiscIntNeverNeededParam
  Discharge_Current_Limit : Gain  Gain=G.dcdc.Iref_limit_A
  Duty_AW_Error : Sum  Inputs=+-
  Duty_AW_Gain : Gain  Gain=G.dcdc.Kaw_i_per_s
  Duty_Command_Sum : Sum  Inputs=+++
  Duty_Integrator_Input : Sum
  Duty_Limit : Saturate  UpperLimit=G.dcdc.duty_max  LowerLimit=G.dcdc.duty_min
  Duty_to_PS : nesl_utility/Simulink-PS Converter  PhysicalDomain=network_engine_domain  SubClassName=ps_input  LeftPortType=input  RightPortType=output  PseudoPeriodic=off  Frequencies=[]  NoiseDistribution=none  NoiseParameters=[]  Unit=1  AffineConversion=off  FilteringAndDerivatives=zero  SimscapeFilterOrder=1  InputFilterTimeConstant=0.001  UdotUserProvided=0
  Hardware_Current_Limit : Saturate  UpperLimit=G.dcdc.Iref_limit_A  LowerLimit=-G.dcdc.Iref_limit_A
  Idc_Filter : StateSpace  A=-1/G.dcdc.current_sensor_s  B=1/G.dcdc.current_sensor_s  D=0  InitialCondition=G.dcdc.Iref_initial_A
  Operating duty : Fcn  Expr=u/(1200+u)
  P_DC_Feedforward_Filter : StateSpace  A=-1/G.dcdc.power_ff_filter_s  B=1/G.dcdc.power_ff_filter_s  D=0  InitialCondition=0
  P_to_Battery_Current_FF : Gain  Gain=1/(G.dc.Vbattery_V*G.dc.dcdc_efficiency_pct/100)
  SOC_Charge_Allowed : simulink/Logic and Bit Operations/Compare To Constant  relop=<  const=G.bess.SOC_max  OutDataTypeStr=boolean
  SOC_Discharge_Allowed : simulink/Logic and Bit Operations/Compare To Constant  relop=>  const=G.bess.SOC_min  OutDataTypeStr=boolean
  Vdc_AW_Error : Sum  Inputs=+-
  Vdc_AW_Gain : Gain  Gain=G.dcdc.Kaw_v_per_s
  Vdc_Error : Sum  Inputs=+-
  Vdc_Filter : StateSpace  A=-1/G.control.Vdc_filter_s  B=1/G.control.Vdc_filter_s  D=0  InitialCondition=G.dc.Vdc_ref_V
  Vdc_For_Modulation : Saturate  UpperLimit=2000  LowerLimit=500
  Vdc_Integrator_Input : Sum
  Vdc_Ki : Gain  Gain=G.dcdc.Kiv_A_per_Vs
  Vdc_Kp : Gain  Gain=G.dcdc.Kpv_A_per_V
  Vdc_PI_Integrator : DiscreteIntegrator  SampleTime=100e-6  ICPrevOutput=DiscIntNeverNeededParam  ICPrevScaledInput=DiscIntNeverNeededParam
  Vdc_Reference : Constant  Value=G.dc.Vdc_ref_V
  output : PMIOPort  Side=Right
  tag scope: R8_02_Bidirectional_DC_DC_Control_p1_signal=global, R8_02_Bidirectional_DC_DC_Control_p2_signal=global, R8_02_Bidirectional_DC_DC_Control_p3_signal=global
  wires:
  Duty_AW_Gain/1 -> Duty_Integrator_Input/2
  Duty_Limit/1 -> [R8_02_Bidirectional_DC_DC_Control_p2_signal], Duty_AW_Error/1, Duty_to_PS/1  "duty_pu"
  Duty_Integrator_Input/1 -> DC_Current_PI_Integrator/1
  DC_Current_Error/1 -> DC_Current_Ki/1, DC_Current_Kp/1
  Idc_Filter/1 -> DC_Current_Error/2
  Discharge_Current_Limit/1 -> DC_Current_Limit/1
  Vdc_Ki/1 -> Vdc_Integrator_Input/1
  SOC_Charge_Allowed/1 -> Charge_Current_Limit/1
  DC_Current_Limit/1 -> [R8_02_Bidirectional_DC_DC_Control_p3_signal], DC_Current_Error/1, Vdc_AW_Error/1
  [R8_01_Battery_and_DC_Link_p2_signal] -> Idc_Filter/1
  Vdc_AW_Error/1 -> Vdc_AW_Gain/1
  Charge_Current_Limit/1 -> DC_Current_Limit/3
  Hardware_Current_Limit/1 -> DC_Current_Limit/2  "Ibat_ref_A"
  Vdc_Integrator_Input/1 -> Vdc_PI_Integrator/1
  Battery_Current_Reference/1 -> Hardware_Current_Limit/1, Vdc_AW_Error/2
  DC_Current_PI_Integrator/1 -> Duty_Command_Sum/2
  SOC_Discharge_Allowed/1 -> Discharge_Current_Limit/1
  Vdc_PI_Integrator/1 -> Battery_Current_Reference/2
  [R8_04_PCS_Filter_and_Transformer_p1_signal] -> P_DC_Feedforward_Filter/1
  Vdc_For_Modulation/1 -> [R8_02_Bidirectional_DC_DC_Control_p1_signal]
  [R8_SOC_FOR_PROTECTION] -> SOC_Discharge_Allowed/1, SOC_Charge_Allowed/1
  Vdc_Error/1 -> Vdc_Kp/1, Vdc_Ki/1
  Duty_AW_Error/1 -> Duty_AW_Gain/1
  Vdc_AW_Gain/1 -> Vdc_Integrator_Input/2
  Vdc_Reference/1 -> Vdc_Error/1
  [R8_01_Battery_and_DC_Link_p1_signal] -> Vdc_Filter/1
  DC_Current_Ki/1 -> Duty_Integrator_Input/1
  P_DC_Feedforward_Filter/1 -> P_to_Battery_Current_FF/1
  Vdc_Kp/1 -> Battery_Current_Reference/1
  DC_Current_Kp/1 -> Duty_Command_Sum/1
  P_to_Battery_Current_FF/1 -> Battery_Current_Reference/3
  Duty_Command_Sum/1 -> Duty_AW_Error/2, Duty_Limit/1
  Vdc_Filter/1 -> Vdc_For_Modulation/1, Vdc_Error/2, Operating duty/1
  Operating duty/1 -> Duty_Command_Sum/3
  connections:
  Duty_to_PS/RConn1 -- output/RConn1

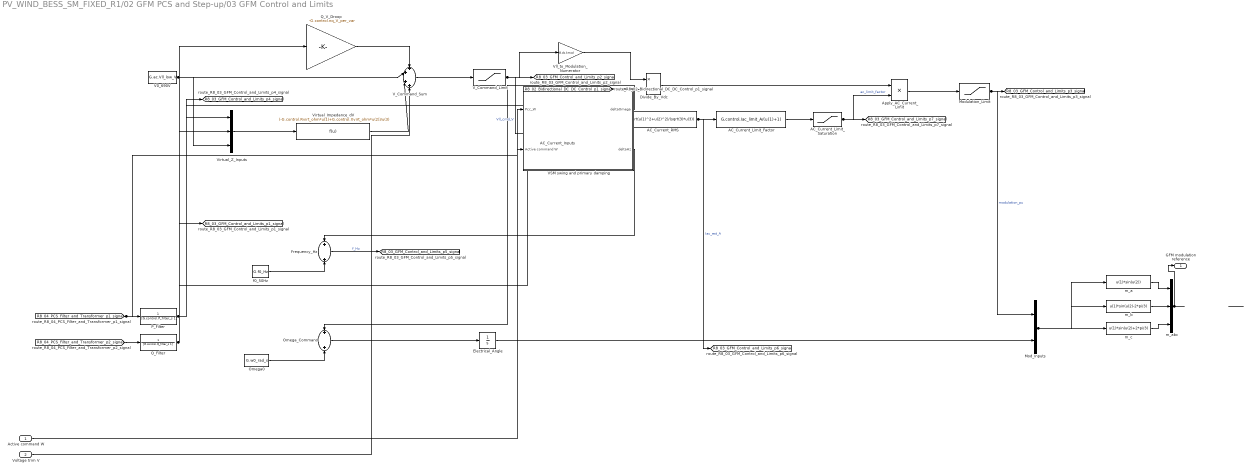
== system PV_WIND_BESS_SM_FIXED_R1/02 GFM PCS and Step-up/03 GFM Control and Limits ==
  Active command W : Inport
  Voltage trim V : Inport  Port=2
  AC_Current_Inputs : Mux  Inputs=3
  AC_Current_Limit_Factor : Fcn  Expr=G.control.Iac_limit_A/(u(1)+1)
  AC_Current_Limit_Saturation : Saturate  UpperLimit=1  LowerLimit=0
  AC_Current_RMS : Fcn  Expr=sqrt(u(1)^2+u(2)^2)/(sqrt(3)*u(3))
  Apply_AC_Current_Limit : Product
  Divide_By_Vdc : Product  Inputs=*/
  Electrical_Angle : Integrator  InitialCondition=pi/6
  Frequency_Hz : Sum
  Mod_Inputs : Mux  Inputs=2
  Modulation_Limit : Saturate  UpperLimit=G.dc.modulation_max  LowerLimit=0
  Omega0 : Constant  Value=G.w0_rad_s
  Omega_Command : Sum
  P_Filter : TransferFcn  Numerator=1  Denominator=[G.control.P_filter_s 1]
  Q_Filter : TransferFcn  Numerator=1  Denominator=[G.control.Q_filter_s 1]
  Q_V_Droop : Gain  Gain=-G.control.nq_V_per_var
  V0_690V : Constant  Value=G.ac.Vll_low_V
  VSM swing and primary damping : Subsystem
  V_Command_Limit : Saturate  UpperLimit=1.10*G.ac.Vll_low_V  LowerLimit=0.90*G.ac.Vll_low_V
  V_Command_Sum : Sum  Inputs=++++
  Virtual_Impedance_dV : Fcn  Expr=(-G.control.Rvirt_ohm*u(1)+G.control.Xvirt_ohm*u(2))/u(3)
  Virtual_Z_Inputs : Mux  Inputs=3
  Vll_to_Modulation_Numerator : Gain  Gain=G.dc.kmod
  f0_50Hz : Constant  Value=G.f0_Hz
  m_a : Fcn  Expr=u(1)*sin(u(2))
  m_abc : Mux  Inputs=3
  m_b : Fcn  Expr=u(1)*sin(u(2)-2*pi/3)
  m_c : Fcn  Expr=u(1)*sin(u(2)+2*pi/3)
  GFM modulation reference : Outport
  tag scope: R8_03_GFM_Control_and_Limits_p1_signal=global, R8_03_GFM_Control_and_Limits_p2_signal=global, R8_03_GFM_Control_and_Limits_p3_signal=global, R8_03_GFM_Control_and_Limits_p4_signal=global, R8_03_GFM_Control_and_Limits_p5_signal=global, R8_03_GFM_Control_and_Limits_p6_signal=global, R8_03_GFM_Control_and_Limits_p7_signal=global
  wires:
  m_abc/1 -> GFM modulation reference/1
  m_c/1 -> m_abc/3
  m_b/1 -> m_abc/2
  Mod_Inputs/1 -> m_a/1, m_b/1, m_c/1
  m_a/1 -> m_abc/1
  Modulation_Limit/1 -> Mod_Inputs/1, [R8_03_GFM_Control_and_Limits_p3_signal]  "modulation_pu"
  AC_Current_Limit_Saturation/1 -> Apply_AC_Current_Limit/2, [R8_03_GFM_Control_and_Limits_p7_signal]  "ac_limit_factor"
  V_Command_Sum/1 -> V_Command_Limit/1
  Divide_By_Vdc/1 -> Apply_AC_Current_Limit/1
  AC_Current_Inputs/1 -> AC_Current_RMS/1
  [R8_02_Bidirectional_DC_DC_Control_p1_signal] -> Divide_By_Vdc/2
  Vll_to_Modulation_Numerator/1 -> Divide_By_Vdc/1
  Apply_AC_Current_Limit/1 -> Modulation_Limit/1
  V_Command_Limit/1 -> Vll_to_Modulation_Numerator/1, AC_Current_Inputs/3, [R8_03_GFM_Control_and_Limits_p2_signal]  "Vll_cmd_V"
  Virtual_Z_Inputs/1 -> Virtual_Impedance_dV/1
  Frequency_Hz/1 -> [R8_03_GFM_Control_and_Limits_p5_signal]  "f_Hz"
  Virtual_Impedance_dV/1 -> V_Command_Sum/3
  Omega0/1 -> Omega_Command/2
  AC_Current_Limit_Factor/1 -> AC_Current_Limit_Saturation/1
  AC_Current_RMS/1 -> AC_Current_Limit_Factor/1, [R8_03_GFM_Control_and_Limits_p6_signal]  "Iac_est_A"
  Q_V_Droop/1 -> V_Command_Sum/1
  f0_50Hz/1 -> Frequency_Hz/2
  P_Filter/1 -> [R8_03_GFM_Control_and_Limits_p4_signal], AC_Current_Inputs/1, Virtual_Z_Inputs/1
  Electrical_Angle/1 -> Mod_Inputs/2
  Omega_Command/1 -> Electrical_Angle/1
  [R8_04_PCS_Filter_and_Transformer_p2_signal] -> Q_Filter/1
  V0_690V/1 -> Virtual_Z_Inputs/3, V_Command_Sum/2
  Q_Filter/1 -> [R8_03_GFM_Control_and_Limits_p1_signal], Virtual_Z_Inputs/2, AC_Current_Inputs/2, Q_V_Droop/1
  [R8_04_PCS_Filter_and_Transformer_p1_signal] -> P_Filter/1, VSM swing and primary damping/1(Pcc_W)
  VSM swing and primary damping/1(deltaOmega) -> Omega_Command/1
  VSM swing and primary damping/2(deltaHz) -> Frequency_Hz/1
  Active command W/1 -> VSM swing and primary damping/2(Active command W)
  Voltage trim V/1 -> V_Command_Sum/4
  connections:
  ?
